simulink model "inverterfullbridge_BIPOLAR_with_rl_load"  (R2023b)
settings: Solver=FixedStepAuto  StartTime=0.0  StopTime=0.1  FixedStep=1/50000  RelTol=1e-3
libraries: spsIGBTDiodeLib x4, spsCurrentMeasurementLib x1, spsDCVoltageSourceLib x1, simulink x1, spsSeriesRLCBranchLib x1, spsVoltageMeasurementLib x1, sps_lib x1
settings Model: Creator=junio  LastModifiedBy=Anuj
settings DataIOCC: ReturnWorkspaceOutputs=off

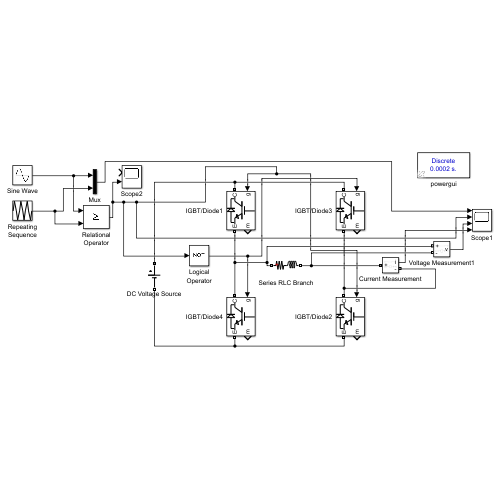
[thumbnail: Simulink's stored preview of the top-level diagram]
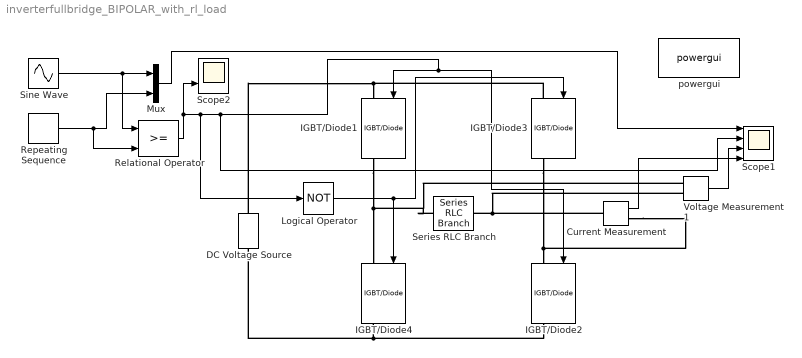
== system inverterfullbridge_BIPOLAR_with_rl_load ==
  Current Measurement : spsCurrentMeasurementLib/Current Measurement  PhasorSimulation=off  OutputType=Complex  PSBequivalent=0
  DC Voltage Source : spsDCVoltageSourceLib/DC Voltage Source  Amplitude=24  Measurements=Voltage
  IGBT/Diode{1..4} (4 alike) : spsIGBTDiodeLib/IGBT//Diode  Ron=1e-3  Rs=1e5  Cs=inf  Measurements=on
  Logical Operator : Logic  Operator=NOT  AllPortsSameDT=off  OutDataTypeStr=boolean
  Mux : Mux  Inputs=2
  Relational Operator : RelationalOperator  OutDataTypeStr=boolean  RndMeth=Simplest  InputSameDT=off
  Repeating Sequence : simulink/Sources/Repeating Sequence  rep_seq_t=[0 0.25 .5 .75 1]*(1/500)  rep_seq_y=[0 1 0 -1 0]
  Scope1 : Scope  NumInputPorts=4
  Scope2 : Scope  NumInputPorts=2
  Series RLC Branch : spsSeriesRLCBranchLib/Series RLC Branch  LConnTagsString=__new0  RConnTagsString=__new0  BranchType=RL  Resistance=10  Inductance=500e-3  SetiL0=off  InitialCurrent=0  Capacitance=1e-6  Setx0=off  InitialVoltage=0  Measurements=None
  Sine Wave : Sin  Frequency=2*pi*50  SampleTime=0
  Voltage Measurement1 : spsVoltageMeasurementLib/Voltage Measurement  PhasorSimulation=off  OutputType=Complex  PSBequivalent=0
  powergui : sps_lib/powergui  Priority=1  SimulationMode=Discrete  SampleTime=1/5000  frequency=60  Iterations=50  frequencyindice=0  Pbase=100e6  ErrMax=1e-4  UnitsV=kV  UnitsW=MW  buscounter=0  FunctionMessages=off  echomessages=off  EnableUseOfTLC=off  CurrentSourceSwitches=off  DisableSnubberDevices=off  DisableRonSwitches=off  DisableVfSwitches=off  DisplayEquations=off  AutomaticDiscreteSolvers=off  SolverType=Tustin/Backward Euler (TBE)  Interpol=off  ExternalGateDelay=off  methode=off  Ts=100  x0status=blocks  SPID=on  SwTol=0  HookPort=off  NonlinearTolerance=1e-4  nMaxIteration=100  ContinueOnMaxIteration=off  RestoreLinks=warning  ResistiveCurrentMeasurement=off  Frange=[0:2:500]  Ylog=off  Xlog=on  ShowGrid=off  save=off  variable=ZData  structure=0  ZoomFFT=off  StartTime=0.0  cycles=1  DisplayStyle=1  fundamental=60  FreqAxis=off  MaxFrequency=1000  frequencyindicesteady=1  RmsSteady=1  display=off
  wires:
  Voltage Measurement1/1 -> Scope1/3
  Sine Wave/1 -> Mux/1, Relational Operator/1
  Repeating Sequence/1 -> Relational Operator/2, Mux/2
  Mux/1 -> Scope1/1
  Logical Operator/1 -> IGBT/Diode3/1, IGBT/Diode4/1
  Relational Operator/1 -> Logical Operator/1, Scope1/2, IGBT/Diode2/1, IGBT/Diode1/1, Scope2/2
  Current Measurement/1 -> Scope1/4
  connections:
  IGBT/Diode3/RConn1 -- Current Measurement/RConn1 -- IGBT/Diode2/LConn1
  IGBT/Diode1/RConn1 -- Voltage Measurement1/LConn1 -- Series RLC Branch/LConn1 -- IGBT/Diode4/LConn1
  IGBT/Diode4/RConn1 -- IGBT/Diode2/RConn1 -- DC Voltage Source/LConn1
  DC Voltage Source/RConn1 -- IGBT/Diode3/LConn1 -- IGBT/Diode1/LConn1
  Current Measurement/LConn1 -- Voltage Measurement1/LConn2 -- Series RLC Branch/RConn1
